simulink model "modelManipulatorSimulink"  (R2026b)
settings: Solver=ode113  StopTime=50  MaxStep=1e-2  RelTol=1e-5
settings Model: Creator=mikolaj  LastModifiedBy=mikolaj

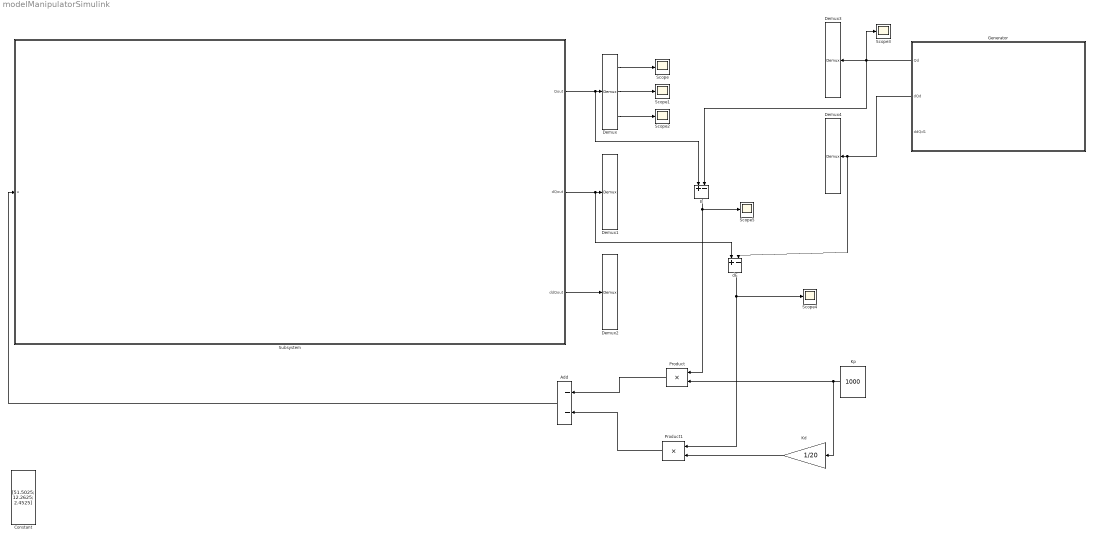
== system modelManipulatorSimulink ==
  Add : Sum  Inputs=--
  Constant : Constant  Value=[51.5025; 12.2625; 2.4525]
  Demux{,1..4} (5 alike) : Demux  Outputs=3
  E : Sum  Inputs=+-
  Generator : Subsystem
  Kd : Gain  Gain=1/20
  Kp : Constant  Value=1000
  Product : Product
  Product1 : Product
  Scope{,1..5} (6 alike) : Scope
      Scope settings: ActiveDisplayYMinimum=-3.6901502323712241  ActiveDisplayYMaximum=0.56019317448146333  DataLoggingVariableName=ScopeData6
      Scope1 settings: ActiveDisplayYMinimum=-17.119601760443715  ActiveDisplayYMaximum=11.561812321736413  DataLoggingVariableName=ScopeData7
      Scope2 settings: ActiveDisplayYMinimum=-14.486850177263117  ActiveDisplayYMaximum=22.074941581395308  DataLoggingVariableName=ScopeData8
      Scope3 settings: ActiveDisplayYMinimum=-0.41136407309554235  ActiveDisplayYMaximum=2.2934586048809025  DataLoggingVariableName=ScopeData15
      Scope4 settings: ActiveDisplayYMinimum=-533.06361578090639  ActiveDisplayYMaximum=527.91065192586041  DataLoggingVariableName=ScopeData16
      Scope5 settings: ActiveDisplayYMinimum=-4.4687166832081218  ActiveDisplayYMaximum=4.1654939973776868  DataLoggingVariableName=ScopeData17
  Subsystem : Subsystem
  dE : Sum  Inputs=+-
  wires:
  Subsystem/1(Qout) -> E/1, Demux/1
  Subsystem/2(dQout) -> dE/1, Demux1/1
  Subsystem/3(ddQout) -> Demux2/1
  Demux/1 -> Scope/1
  Demux/2 -> Scope1/1
  Demux/3 -> Scope2/1
  Generator/1(Qd) -> Scope3/1, Demux3/1, E/2
  Generator/2(dQd) -> dE/2, Demux4/1
  Kd/1 -> Product1/2
  Kp/1 -> Product/2, Kd/1
  dE/1 -> Product1/1, Scope4/1
  E/1 -> Product/1, Scope5/1
  Product/1 -> Add/1
  Product1/1 -> Add/2
  Add/1 -> Subsystem/1(u)

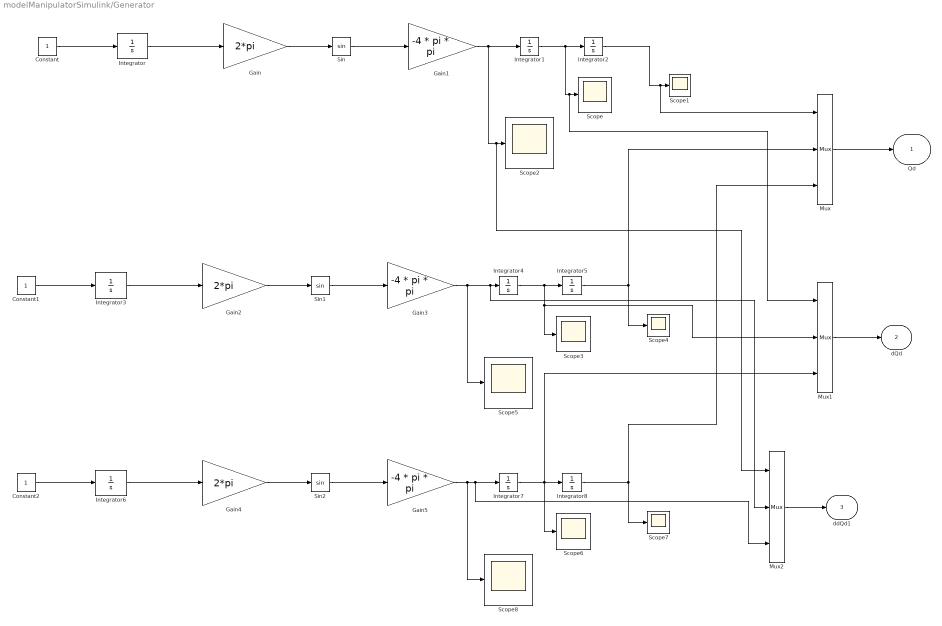
== system modelManipulatorSimulink/Generator ==
  Constant : Constant
  Constant1 : Constant
  Constant2 : Constant
  Gain : Gain  Gain=2*pi
  Gain1 : Gain  Gain=-4 * pi * pi
  Gain2 : Gain  Gain=2*pi
  Gain3 : Gain  Gain=-4 * pi * pi
  Gain4 : Gain  Gain=2*pi
  Gain5 : Gain  Gain=-4 * pi * pi
  Integrator : Integrator
  Integrator1 : Integrator  InitialCondition=2*pi
  Integrator2 : Integrator  InitialCondition=1
  Integrator3 : Integrator
  Integrator4 : Integrator  InitialCondition=2*pi
  Integrator5 : Integrator  InitialCondition=1
  Integrator6 : Integrator
  Integrator7 : Integrator  InitialCondition=2*pi
  Integrator8 : Integrator  InitialCondition=1
  Mux : Mux  Inputs=3
  Mux1 : Mux  Inputs=3
  Mux2 : Mux  Inputs=3
  Scope{,1..8} (9 alike) : Scope
      Scope settings: ActiveDisplayYMinimum=-7.8539688359124664  ActiveDisplayYMaximum=7.8539802119675919  DataLoggingVariableName=ScopeData3
      Scope1 settings: ActiveDisplayYMinimum=-0.24999710016798737  ActiveDisplayYMaximum=2.2499971001724131  DataLoggingVariableName=ScopeData4
      Scope2 settings: ActiveDisplayYMinimum=-49.347932658064352  ActiveDisplayYMaximum=49.34793265806438  DataLoggingVariableName=ScopeData5
      Scope3 settings: ActiveDisplayYMinimum=-7.8539688359124664  ActiveDisplayYMaximum=7.8539802119675919  DataLoggingVariableName=ScopeData9
      Scope4 settings: ActiveDisplayYMinimum=-0.24999710016798737  ActiveDisplayYMaximum=2.2499971001724131  DataLoggingVariableName=ScopeData10
      Scope5 settings: ActiveDisplayYMinimum=-49.347932658064352  ActiveDisplayYMaximum=49.34793265806438  DataLoggingVariableName=ScopeData11
      Scope6 settings: ActiveDisplayYMinimum=-7.8539688359124664  ActiveDisplayYMaximum=7.8539802119675919  DataLoggingVariableName=ScopeData12
      Scope7 settings: ActiveDisplayYMinimum=-0.24999710016798737  ActiveDisplayYMaximum=2.2499971001724131  DataLoggingVariableName=ScopeData13
      Scope8 settings: ActiveDisplayYMinimum=-49.347932658064352  ActiveDisplayYMaximum=49.34793265806438  DataLoggingVariableName=ScopeData14
  Sin : Trigonometry
  Sin1 : Trigonometry
  Sin2 : Trigonometry
  Qd : Outport
  dQd : Outport  Port=2
  ddQd1 : Outport  Port=3
  wires:
  Constant/1 -> Integrator/1
  Integrator/1 -> Gain/1
  Gain/1 -> Sin/1
  Sin/1 -> Gain1/1
  Gain1/1 -> Mux2/1, Scope2/1, Integrator1/1
  Integrator1/1 -> Mux1/1, Scope/1, Integrator2/1
  Integrator2/1 -> Mux/1, Scope1/1
  Integrator4/1 -> Mux1/2, Scope3/1, Integrator5/1
  Constant1/1 -> Integrator3/1
  Gain3/1 -> Scope5/1, Mux2/2, Integrator4/1
  Integrator3/1 -> Gain2/1
  Sin1/1 -> Gain3/1
  Gain2/1 -> Sin1/1
  Integrator5/1 -> Mux/2, Scope4/1
  Sin2/1 -> Gain5/1
  Integrator6/1 -> Gain4/1
  Constant2/1 -> Integrator6/1
  Gain5/1 -> Scope8/1, Mux2/3, Integrator7/1
  Integrator8/1 -> Mux/3, Scope7/1
  Integrator7/1 -> Mux1/3, Scope6/1, Integrator8/1
  Gain4/1 -> Sin2/1
  Mux/1 -> Qd/1
  Mux2/1 -> ddQd1/1
  Mux1/1 -> dQd/1

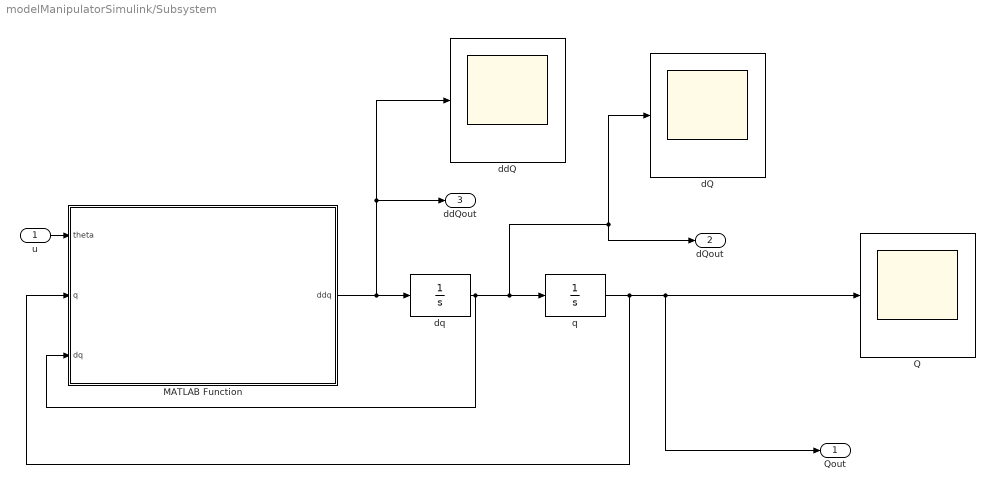
== system modelManipulatorSimulink/Subsystem ==
  u : Inport
  MATLAB Function : MATLAB Function  TreatAsAtomicUnit=on
  Q : Scope
      settings: ActiveDisplayYMinimum=-82.520337529201385  ActiveDisplayYMaximum=52.171009313163665
  dQ : Scope
      settings: ActiveDisplayYMinimum=-82.520337529201385  ActiveDisplayYMaximum=52.171009313163665
  ddQ : Scope
      settings: ActiveDisplayYMinimum=-82.520337529201385  ActiveDisplayYMaximum=52.171009313163665  DataLoggingVariableName=ScopeData2
  dq : Integrator  InitialCondition=[1; 1; 1]
  q : Integrator  InitialCondition=[0; 0; 0]
  Qout : Outport
  dQout : Outport  Port=2
  ddQout : Outport  Port=3
  wires:
  MATLAB Function/1(ddq) -> ddQ/1, ddQout/1, dq/1
  dq/1 -> MATLAB Function/3(dq), dQout/1, dQ/1, q/1
  q/1 -> MATLAB Function/2(q), Qout/1, Q/1
  u/1 -> MATLAB Function/1(theta)

== matlab function modelManipulatorSimulink/Subsystem/MATLAB Function ==
  data: theta input; ddq output; q input; dq input
function ddq = dynamika(theta, q ,dq)


l1 = 0.5; l2 = 0.5; l3 = 0.5;
m1 = 10; m2 = 2; m3 = 1;
g = 9.81;
q1 = q(1); q2 = q(2); q3 = q(3);
dq1 = dq(1); dq2 = dq(2); dq3 = dq(3);


% Q11 = 1/3 * m1 * l1^2 + m2*l1^2 + 1/3 * m2 * l2^2 + m2*l1*l2*cos(q2) + 1/3 * m3 *l3^2 + m3*(l1^2 + l2^2 + l2*l3*cos(q3) + 2*l1*l2*cos(q2)+l1*l3*cos(q2+q3))  ;
% Q12 = 1/3 * m2 * l2^2 + 1/2 * m2 * l1 * l2 * cos(q2) + 1/3 * m3 * l3^2 + m3*(l2^2+l2*l3*cos(q3)+l1*l2*cos(q2)+1/2*l1*l3*cos(q2+q3));
% Q13 = 1/3 * m3 * l3^2 + 1/2 * m3 * (l2*l3*cos(q3) + l1*l3*cos(q2+q3));
% Q22 = 1/3 * m2 * l2^2 + 1/3 * m3 * l3^2 + m3*(l2*l3*cos(q3) + l2^2);
% Q23 = 1/3 * m3 * l3^2 + 1/2 * m3 * l2 * l3 * cos(q3);
% Q33 = 1/3 * m3 * l3^2;
% M = [Q11 Q12 Q13;
%     Q12 Q22 Q23;
%     Q13 Q23 Q33];
% 
% C11 = -1/2 * dq2 * (m2*l1*l2*sin(q2) + 2*m3*l1*l2*sin(q2) + m3*l1*l3*sin(q2+q3)) - 1/2*dq3*(m3*l2*l3*sin(q3) + m3*l1*l3*sin(q2+q3));
% C12 = -1/2 * (dq1 + dq2) * (m2*l1*l2*sin(q2) + 2*m3*l1*l2*sin(q2) + m3*l1*l3*sin(q2+q3)) - 1/2 * dq3 * (m2*l2*l3*sin(q3) + m3*l1*l3*sin(q2+q3));
% C13 = -1/2 * (dq1 + dq2 + dq3) * (m3*l2*l3*sin(q3) + m3*l1*l3*sin(q2+q3));
% C21 = 1/2 * dq1 * (m2*l1*l2*sin(q2) + 2*m3*l1*l2*sin(q2) + m3*l1*l3*sin(q2+q3)) - 1/2*dq3*m3*l2*l3*sin(q3);
% C22 = -1/2 * dq3 * m3 * l2 * l3 * sin(q3);
% C23 = -1/2 *(dq1 + dq2 + dq3)*m3*l2*l3*sin(q3);
% C31 = 1/2 * dq1 * (m3*l2*l3*sin(q3) + m3*l1*l3*sin(q2+q3)) + 1/2 * dq2*m3*l2*l3*sin(q3);
% C32 = 1/2 * (dq1 + dq2)*m3*l2*l3*sin(q3);
% 
% C = [C11 C12 C13;
%      C21 C22 C23;
%      C31 C32 0];
% 
% D1 = 1/2 * g * ( (m1 + 2*m2 + 2*m3)*l1*cos(q1) + (m2 + 2*m3)*l2*cos(q1+q2) + m3*l3*cos(q1+q2+q3));
% D2 = 1/2 * g * ( (m2 + 2*m3)*l2*cos(q1+q2) + m3*l3*cos(q1+q2+q3));
% D3 = 1/2 * g * m3*l3*cos(q1+q2+q3);
% 
% D = [D1;
%      D2;
%      D3];

Q11 = cos(q2 + q3)/4 + cos(q2) + cos(q3)/4 + 25/12;
Q12 = cos(q2 + q3)/8 + cos(q2)/2 + cos(q3)/4 + 1/2;
Q13 = cos(q2 + q3)/8 + cos(q3)/8 + 1/12;
Q22 = cos(q3)/4 + 1/2;
Q23 = cos(q3)/8 + 1/12;
Q33 = 1/12;
M = [Q11 Q12 Q13;
    Q12 Q22 Q23;
    Q13 Q23 Q33];
% 
% C11 = - (dq2*(sin(q2 + q3)/4 + sin(q2)))/2 - (dq3*(sin(q2 + q3)/4 + sin(q3)/4))/2;
% C12 = (dq1*(sin(q2 + q3)/4 + sin(q2)))/2 - (dq3*sin(q3))/8;
% C13 = (dq1*(sin(q2 + q3)/4 + sin(q3)/4))/2 + (dq2*sin(q3))/8;
% C21 = - (dq3*(sin(q2 + q3)/4 + sin(q3)/2))/2 - (sin(q2 + q3)/4 + sin(q2))*(dq1/2 + dq2/2);
% C22 = -(dq3*sin(q3))/8;
% C23 = (sin(q3)*(dq1/2 + dq2/2))/4;
% C31 = -(sin(q2 + q3)/4 + sin(q3)/4)*(dq1/2 + dq2/2 + dq3/2);
% C32 = -(sin(q3)*(dq1/2 + dq2/2 + dq3/2))/4;
% C33 = 0;

C11 = - (dq2*(sin(q2 + q3)/4 + sin(q2)))/2 - (dq3*(sin(q2 + q3)/4 + sin(q3)/4))/2;
C12 = - (dq3*(sin(q2 + q3)/4 + sin(q3)/4))/2 - (sin(q2 + q3)/4 + sin(q2))*(dq1/2 + dq2/2);
C13 = -(sin(q2 + q3)/4 + sin(q3)/4)*(dq1/2 + dq2/2 + dq3/2);
C21 = (dq1*(sin(q2 + q3)/4 + sin(q2)))/2 - (dq3*sin(q3))/8;
C22 = -(dq3*sin(q3))/8;
C23 = -(sin(q3)*(dq1/2 + dq2/2 + dq3/2))/4;
C31 = (dq1*(sin(q2 + q3)/4 + sin(q3)/4))/2 + (dq2*sin(q3))/8;
C32 = (sin(q3)*(dq1/2 + dq2/2))/4;
C33 = 0;

C = [C11 C12 C13;
    C21 C22 C23;
    C31 C32 C33];

D1 = (981*cos(q1 + q2 + q3))/400 + (981*cos(q1 + q2))/100 + (981*cos(q1))/25;
D2 = (981*cos(q1 + q2 + q3))/400 + (981*cos(q1 + q2))/100;
D3 = (981*cos(q1 + q2 + q3))/400;

D = [D1;
    D2;
    D3];

ddq = M \ (theta - C*dq - D);
